simulink subsystem "MagneticField"  (R2024b)
settings: Solver=VariableStepAuto  StartTime=0.0  StopTime=10.0  RelTol=1e-3
undefined symbols (not defined in the file): orbit
settings Model: Creator=marco  LastModifiedBy=ferru

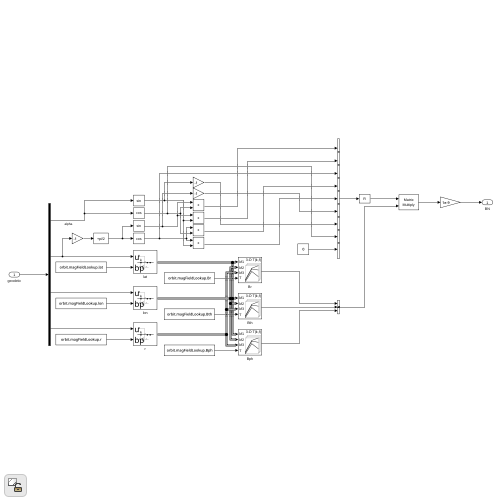
[thumbnail: Simulink's stored preview of the top-level diagram]
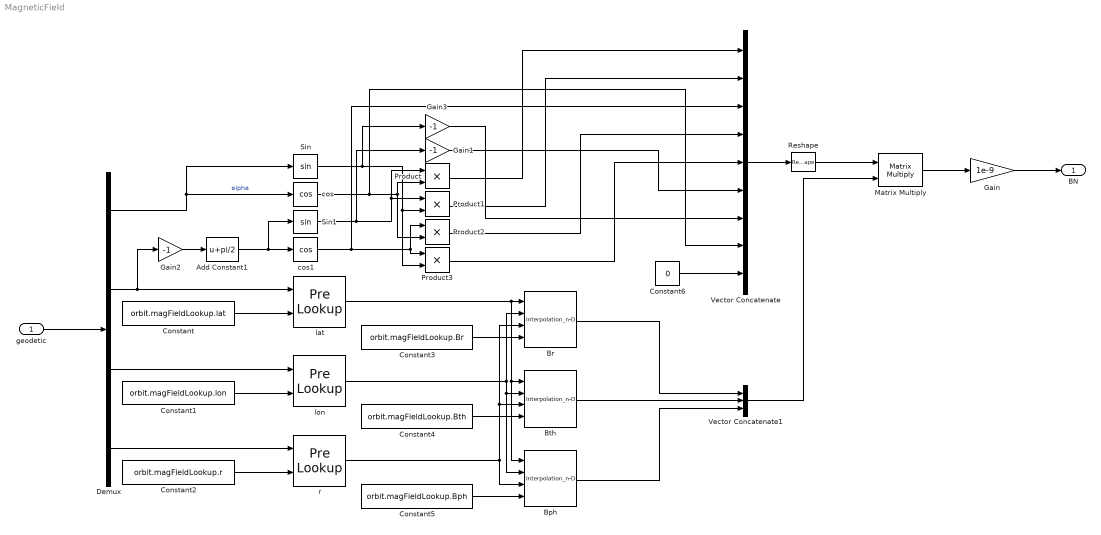
== system MagneticField ==
  geodetic : Inport
  Add Constant1 : Bias  Bias=pi/2  SaturateOnIntegerOverflow=off
  Bph : Interpolation_n-D  NumberOfTableDimensions=3  TableSource=Input port  ExtrapMethod=Clip  RequireIndexFractionAsBus=on  InternalRulePriority=Speed
      settings: InputPortMap=u0,u1,u2,p2
  Br : Interpolation_n-D  NumberOfTableDimensions=3  TableSource=Input port  ExtrapMethod=Clip  RequireIndexFractionAsBus=on  InternalRulePriority=Speed
      settings: InputPortMap=u0,u1,u2,p2
  Bth : Interpolation_n-D  NumberOfTableDimensions=3  TableSource=Input port  ExtrapMethod=Clip  RequireIndexFractionAsBus=on  InternalRulePriority=Speed
      settings: InputPortMap=u0,u1,u2,p2
  Constant : Constant  Value=orbit.magFieldLookup.lat
  Constant1 : Constant  Value=orbit.magFieldLookup.lon
  Constant2 : Constant  Value=orbit.magFieldLookup.r
  Constant3 : Constant  Value=orbit.magFieldLookup.Br
  Constant4 : Constant  Value=orbit.magFieldLookup.Bth
  Constant5 : Constant  Value=orbit.magFieldLookup.Bph
  Constant6 : Constant  Value=0
  Demux : Demux
  Gain : Gain  Gain=1e-9
  Gain1 : Gain  Gain=-1
  Gain2 : Gain  Gain=-1
  Gain3 : Gain  Gain=-1
  Matrix Multiply : Product  Multiplication=Matrix(*)
  Product{,1..3} (4 alike) : Product
  Reshape : Reshape  OutputDimensionality=Customize  OutputDimensions=[3, 3]
  Sin : Trigonometry
  Sin1 : Trigonometry
  Vector Concatenate : Concatenate  NumInputs=9
  Vector Concatenate1 : Concatenate  NumInputs=3  Mode=Multidimensional array
  cos : Trigonometry  Operator=cos
  cos1 : Trigonometry  Operator=cos
  lat : PreLookup  BreakpointsDataSource=Input port  BreakpointsData=[10:10:110]  OutputSelection=Index and fraction as bus  ExtrapMethod=Linear
      settings: InputPortMap=u0,p1
  lon : PreLookup  BreakpointsDataSource=Input port  BreakpointsData=[10:10:110]  OutputSelection=Index and fraction as bus  ExtrapMethod=Linear
      settings: InputPortMap=u0,p1
  r : PreLookup  BreakpointsDataSource=Input port  BreakpointsData=[10:10:110]  OutputSelection=Index and fraction as bus  ExtrapMethod=Linear
      settings: InputPortMap=u0,p1
  BN : Outport
  wires:
  geodetic/1 -> Demux/1
  Matrix Multiply/1 -> Gain/1
  Gain/1 -> BN/1
  lat/1 -> Br/1, Bth/1, Bph/1
  lon/1 -> Br/2, Bth/2, Bph/2
  r/1 -> Bph/3, Bth/3, Br/3
  Demux/2 -> lat/1, Gain2/1
  Demux/3 -> lon/1
  Demux/4 -> r/1
  Constant/1 -> lat/2
  Constant1/1 -> lon/2
  Constant2/1 -> r/2
  Constant4/1 -> Bth/4
  Constant3/1 -> Br/4
  Constant5/1 -> Bph/4
  Demux/1 -> cos/1, Sin/1  "alpha"
  Gain2/1 -> Add Constant1/1
  Add Constant1/1 -> cos1/1, Sin1/1
  cos/1 -> Product2/2, Product/2, Vector Concatenate/8
  Sin1/1 -> Product1/1, Product/1, Gain1/1
  Sin/1 -> Product1/2, Product3/2, Gain3/1
  cos1/1 -> Vector Concatenate/3, Product2/1, Product3/1
  Constant6/1 -> Vector Concatenate/9
  Product1/1 -> Vector Concatenate/2
  Product/1 -> Vector Concatenate/1
  Product2/1 -> Vector Concatenate/4
  Product3/1 -> Vector Concatenate/5
  Gain1/1 -> Vector Concatenate/6
  Gain3/1 -> Vector Concatenate/7
  Vector Concatenate/1 -> Reshape/1
  Reshape/1 -> Matrix Multiply/1
  Bth/1 -> Vector Concatenate1/2
  Br/1 -> Vector Concatenate1/1
  Bph/1 -> Vector Concatenate1/3
  Vector Concatenate1/1 -> Matrix Multiply/2
